simulink model "Stufe2_Laengsdyn1DOF"  (R2026b)
settings: Solver=ode45  StopTime=310  MaxStep=1  RelTol=1e-6
undefined symbols (not defined in the file or in its folder): PAR_Ach_AbstHi_f64, PAR_Lng_BeiwLuft_f64, PAR_Lng_BeiwRoll_f64, PAR_Lng_BeschlErde_f64, PAR_Lng_DichteLuft_f64, PAR_Lng_GeschwStart_f64, PAR_Lng_MasseFzg_f64, PAR_Lng_Stirnfl_f64
libraries: autolibshared x1, simulink x1

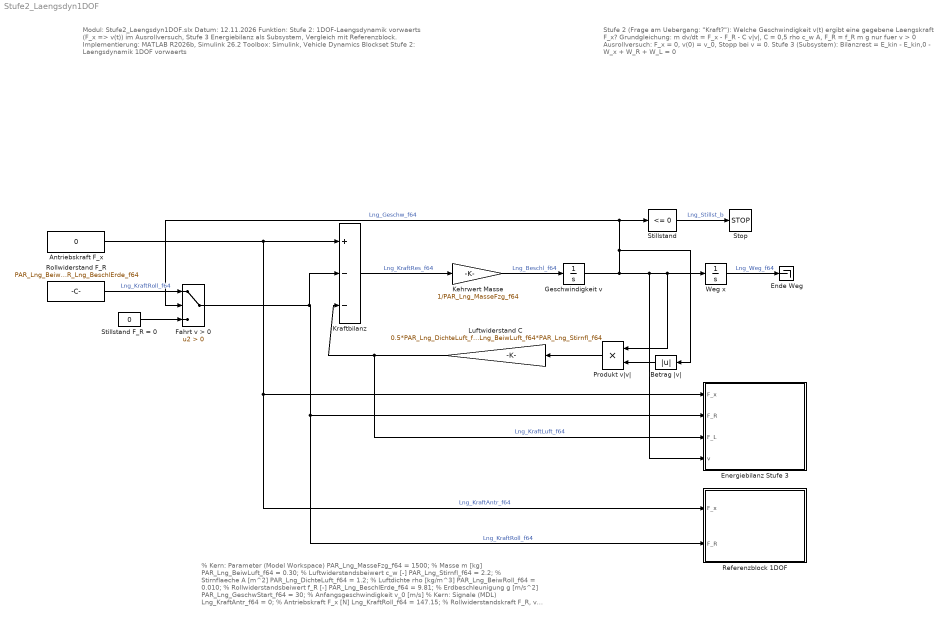
== system Stufe2_Laengsdyn1DOF ==
  note: % Kern: Parameter (Model Workspace)
      | PAR_Lng_MasseFzg_f64 = 1500; % Masse m [kg]
      | PAR_Lng_BeiwLuft_f64 = 0.30; % Luftwiderstandsbeiwert c_w [-]
      | PAR_Lng_Stirnfl_f64 = 2.2; % Stirnflaeche A [m^2]
      | PAR_Lng_DichteLuft_f64 = 1.2; % Luftdichte rho [kg/m^3]
      | PAR_Lng_BeiwRoll_f64 = 0.010; % Rollwiderstandsbeiwert f_R [-]
      | PAR_Lng_BeschlErde_f64 = 9.81; % Erdbeschleunigung g [m/s^2]
      | PAR_Lng_GeschwStart_f64 = 30; % Anfangsgeschwindigkeit v_0 [m/s]
      |
      | % Kern: Signale (MDL)
      | Lng_KraftAntr_f64 = 0; % Antriebskraft F_x [N]
      | Lng_KraftRoll_f64 = 147.15; % Rollwiderstandskraft F_R, v > 0 [N]
      | Lng_KraftLuft_f64 = 'C v|v|' ; % Luftwiderstandskraft F_L [N]
      | Lng_KraftRes_f64 = 'F_x - F_R - F_L' ; % resultierende Kraft [N]
      | Lng_Beschl_f64 = 'F_res/m' ; % Beschleunigung a [m/s^2]
      | Lng_Geschw_f64 = '30 -> 0' ; % Geschwindigkeit v, geloggt [m/s]
      | Lng_Weg_f64 = '0 -> 2330.0' ; % Weg x, geloggt [m]
      | Lng_Stillst_b = 'v <= 0' ; % Stillstand -> Stop [-]
  note: Modul: Stufe2_Laengsdyn1DOF.slx
      | Datum: 12.11.2026
      | Funktion: Stufe 2: 1DOF-Laengsdynamik vorwaerts (F_x => v(t)) im Ausrollversuch,
      | Stufe 3 Energiebilanz als Subsystem, Vergleich mit Referenzblock.
      | Implementierung: MATLAB R2026b, Simulink 26.2
      | Toolbox: Simulink, Vehicle Dynamics Blockset
      |
      | Stufe 2: Laengsdynamik 1DOF vorwaerts
  note: Stufe 2 (Frage am Uebergang: "Kraft?"): Welche Geschwindigkeit v(t) ergibt eine gegebene Laengskraft F_x?
      | Grundgleichung: m dv/dt = F_x - F_R - C v|v|, C = 0,5 rho c_w A, F_R = f_R m g nur fuer v > 0
      | Ausrollversuch: F_x = 0, v(0) = v_0, Stopp bei v = 0.
      | Stufe 3 (Subsystem): Bilanzrest = E_kin - E_kin,0 - W_x + W_R + W_L = 0
  Antriebskraft F_x : Constant  Value=0
  Betrag |v| : Abs  SaturateOnIntegerOverflow=off
  Ende Weg : Terminator
  Energiebilanz Stufe 3 : Subsystem
  Fahrt v > 0 : Switch  Criteria=u2 > Threshold  SaturateOnIntegerOverflow=off  InputSameDT=off
  Geschwindigkeit v : Integrator  InitialCondition=PAR_Lng_GeschwStart_f64
  Kehrwert Masse : Gain  Gain=1/PAR_Lng_MasseFzg_f64
  Kraftbilanz : Sum  Inputs=+--
  Luftwiderstand C : Gain  Gain=0.5*PAR_Lng_DichteLuft_f64*PAR_Lng_BeiwLuft_f64*PAR_Lng_Stirnfl_f64
  Produkt v|v| : Product
  Referenzblock 1DOF : Subsystem
  Rollwiderstand F_R : Constant  Value=PAR_Lng_BeiwRoll_f64*PAR_Lng_MasseFzg_f64*PAR_Lng_BeschlErde_f64
  Stillstand : simulink/Logic and Bit Operations/Compare To Zero  relop=<=  OutDataTypeStr=boolean
  Stillstand F_R = 0 : Constant  Value=0
  Stop : Stop
  Weg x : Integrator
  wires:
  Weg x/1 -> Ende Weg/1  "Lng_Weg_f64"
  Produkt v|v|/1 -> Luftwiderstand C/1
  Stillstand/1 -> Stop/1  "Lng_Stillst_b"
  Geschwindigkeit v/1 -> Stillstand/1, Fahrt v > 0/2, Betrag |v|/1, Weg x/1, Produkt v|v|/1, Energiebilanz Stufe 3/4(v)  "Lng_Geschw_f64"
  Kehrwert Masse/1 -> Geschwindigkeit v/1  "Lng_Beschl_f64"
  Kraftbilanz/1 -> Kehrwert Masse/1  "Lng_KraftRes_f64"
  Luftwiderstand C/1 -> Kraftbilanz/3, Energiebilanz Stufe 3/3(F_L)  "Lng_KraftLuft_f64"
  Antriebskraft F_x/1 -> Referenzblock 1DOF/1(F_x), Energiebilanz Stufe 3/1(F_x), Kraftbilanz/1  "Lng_KraftAntr_f64"
  Rollwiderstand F_R/1 -> Fahrt v > 0/1  "Lng_KraftRoll_f64"
  Stillstand F_R = 0/1 -> Fahrt v > 0/3
  Fahrt v > 0/1 -> Referenzblock 1DOF/2(F_R), Energiebilanz Stufe 3/2(F_R), Kraftbilanz/2  "Lng_KraftRoll_f64"
  Betrag |v|/1 -> Produkt v|v|/2

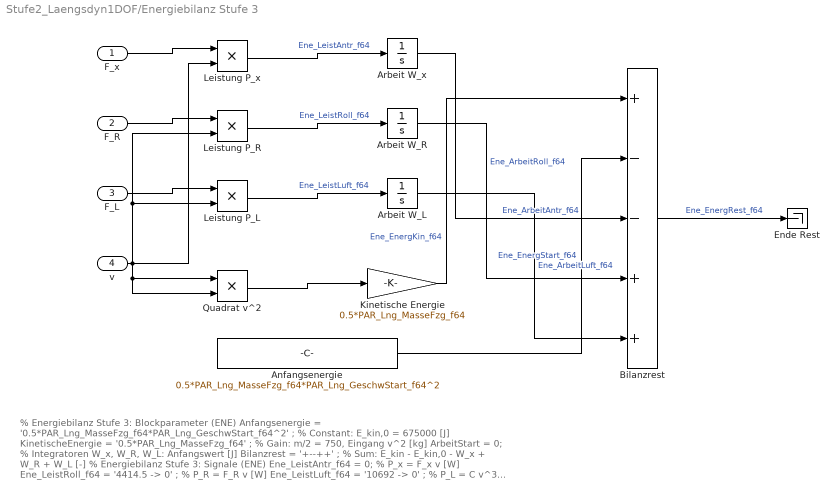
== system Stufe2_Laengsdyn1DOF/Energiebilanz Stufe 3 ==
  note: % Energiebilanz Stufe 3: Blockparameter (ENE)
      | Anfangsenergie = '0.5*PAR_Lng_MasseFzg_f64*PAR_Lng_GeschwStart_f64^2' ; % Constant: E_kin,0 = 675000 [J]
      | KinetischeEnergie = '0.5*PAR_Lng_MasseFzg_f64' ; % Gain: m/2 = 750, Eingang v^2 [kg]
      | ArbeitStart = 0; % Integratoren W_x, W_R, W_L: Anfangswert [J]
      | Bilanzrest = '+--++' ; % Sum: E_kin - E_kin,0 - W_x + W_R + W_L [-]
      |
      | % Energiebilanz Stufe 3: Signale (ENE)
      | Ene_LeistAntr_f64 = 0; % P_x = F_x v [W]
      | Ene_LeistRoll_f64 = '4414.5 -> 0' ; % P_R = F_R v [W]
      | Ene_LeistLuft_f64 = '10692 -> 0' ; % P_L = C v^3 [W]
      | Ene_ArbeitAntr_f64 = 0; % W_x, geloggt [J]
      | Ene_ArbeitRoll_f64 = '0 -> 342857' ; % W_R, geloggt [J]
      | Ene_ArbeitLuft_f64 = '0 -> 332143' ; % W_L, geloggt [J]
      | Ene_EnergKin_f64 = '675000 -> 0' ; % E_kin = m v^2/2 [J]
      | Ene_EnergStart_f64 = 675000; % E_kin,0 [J]
      | Ene_EnergRest_f64 = 'max 3.6e-8' ; % Bilanzrest, Toleranz 0,675 J, geloggt [J]
  F_x : Inport
  F_R : Inport  Port=2
  F_L : Inport  Port=3
  v : Inport  Port=4
  Anfangsenergie : Constant  Value=0.5*PAR_Lng_MasseFzg_f64*PAR_Lng_GeschwStart_f64^2
  Arbeit W_L : Integrator
  Arbeit W_R : Integrator
  Arbeit W_x : Integrator
  Bilanzrest : Sum  Inputs=+--++
  Ende Rest : Terminator
  Kinetische Energie : Gain  Gain=0.5*PAR_Lng_MasseFzg_f64
  Leistung P_L : Product
  Leistung P_R : Product
  Leistung P_x : Product
  Quadrat v^2 : Product
  wires:
  Bilanzrest/1 -> Ende Rest/1  "Ene_EnergRest_f64"
  Arbeit W_L/1 -> Bilanzrest/5  "Ene_ArbeitLuft_f64"
  Arbeit W_R/1 -> Bilanzrest/4  "Ene_ArbeitRoll_f64"
  Arbeit W_x/1 -> Bilanzrest/3  "Ene_ArbeitAntr_f64"
  Anfangsenergie/1 -> Bilanzrest/2  "Ene_EnergStart_f64"
  Kinetische Energie/1 -> Bilanzrest/1  "Ene_EnergKin_f64"
  Quadrat v^2/1 -> Kinetische Energie/1
  Leistung P_L/1 -> Arbeit W_L/1  "Ene_LeistLuft_f64"
  Leistung P_R/1 -> Arbeit W_R/1  "Ene_LeistRoll_f64"
  Leistung P_x/1 -> Arbeit W_x/1  "Ene_LeistAntr_f64"
  F_L/1 -> Leistung P_L/1
  F_R/1 -> Leistung P_R/1
  v/1 -> Quadrat v^2/1, Quadrat v^2/2, Leistung P_R/2, Leistung P_L/2, Leistung P_x/2
  F_x/1 -> Leistung P_x/1

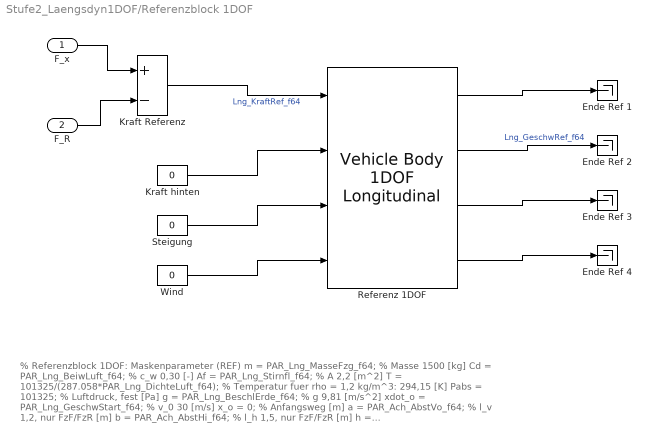
== system Stufe2_Laengsdyn1DOF/Referenzblock 1DOF ==
  note: % Referenzblock 1DOF: Maskenparameter (REF)
      | m = PAR_Lng_MasseFzg_f64; % Masse 1500 [kg]
      | Cd = PAR_Lng_BeiwLuft_f64; % c_w 0,30 [-]
      | Af = PAR_Lng_Stirnfl_f64; % A 2,2 [m^2]
      | T = 101325/(287.058*PAR_Lng_DichteLuft_f64); % Temperatur fuer rho = 1,2 kg/m^3: 294,15 [K]
      | Pabs = 101325; % Luftdruck, fest [Pa]
      | g = PAR_Lng_BeschlErde_f64; % g 9,81 [m/s^2]
      | xdot_o = PAR_Lng_GeschwStart_f64; % v_0 30 [m/s]
      | x_o = 0; % Anfangsweg [m]
      | a = PAR_Ach_AbstVo_f64; % l_v 1,2, nur FzF/FzR [m]
      | b = PAR_Ach_AbstHi_f64; % l_h 1,5, nur FzF/FzR [m]
      | h = PAR_Ach_SchwerpHoehe_f64; % h 0,55, nur FzF/FzR [m]
      | Cl = 0; % Auftriebsbeiwert, aus [-]
      | Cpm = 0; % Nickmomentbeiwert, aus [-]
      | NF = 2; % Raeder vorn [-]
      | NR = 2; % Raeder hinten [-]
      |
      | % Schalter extFMode, extMMode, extTamb, wind3D = off
      | % Referenzblock 1DOF: Blockparameter und Signale (REF)
      | KraftReferenz = '+-' ; % Sum: F_x - F_R -> FwF [-]
      | KraftHinten = 0; % Constant -> FwR [N]
      | Steigung = 0; % Constant -> Grade [deg]
      | Wind = 0; % Constant -> WindX [m/s]
      | Lng_KraftRef_f64 = -147.15; % F_x - F_R am FwF [N]
      | Lng_GeschwRef_f64 = '30 -> 0' ; % v Referenzblock, geloggt [m/s]
      |
      | % Info, FzF, FzR terminiert (Ende Ref 1, 3, 4)
  F_x : Inport
  F_R : Inport  Port=2
  Ende Ref {1..4} (4 alike) : Terminator
  Kraft Referenz : Sum  Inputs=+-
  Kraft hinten : Constant  Value=0
  Referenz 1DOF : autolibshared/Vehicle Body 1DOF Longitudinal  VariantControl=SL  extFMode=off  extMMode=off  extTamb=off  wind3D=off  aMode=2  NF=2  NR=2  m=PAR_Lng_MasseFzg_f64  a=PAR_Ach_AbstVo_f64  b=PAR_Ach_AbstHi_f64  h=PAR_Ach_SchwerpHoehe_f64  Cd=PAR_Lng_BeiwLuft_f64  Cl=0  Cpm=0  Af=PAR_Lng_Stirnfl_f64  x_o=0  xdot_o=PAR_Lng_GeschwStart_f64  Pabs=101325  T=101325/(287.058*PAR_Lng_DichteLuft_f64)  g=PAR_Lng_BeschlErde_f64
      settings: LibrarySourceBlock=vehdynlibeom/Vehicle Body 1DOF Longitudinal
  Steigung : Constant  Value=0
  Wind : Constant  Value=0
  wires:
  F_R/1 -> Kraft Referenz/2
  F_x/1 -> Kraft Referenz/1
  Referenz 1DOF/2 -> Ende Ref 2/1  "Lng_GeschwRef_f64"
  Referenz 1DOF/4 -> Ende Ref 4/1
  Referenz 1DOF/1 -> Ende Ref 1/1
  Wind/1 -> Referenz 1DOF/4
  Kraft Referenz/1 -> Referenz 1DOF/1  "Lng_KraftRef_f64"
  Referenz 1DOF/3 -> Ende Ref 3/1
  Steigung/1 -> Referenz 1DOF/3
  Kraft hinten/1 -> Referenz 1DOF/2
